simulink model "Impl_None"  (R2026b)
settings: Solver=VariableStepAuto
undefined symbols (not defined in the file or in its folder): P, Ts
libraries: fl_lib x7, simulink x1, ee_lib x1
settings Model: Creator=aomar  LastModifiedBy=aomar

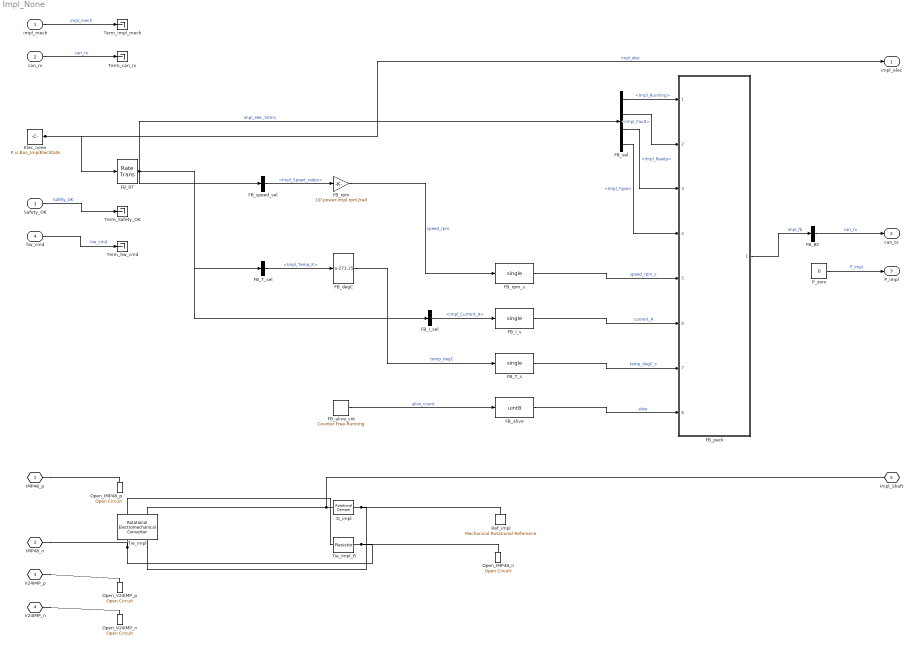
== system Impl_None ==
  impl_mech : Inport  OutDataTypeStr=Bus: Bus_ImplMechState  SampleTime=Ts.ctrl
  can_rx : Inport  Port=2  OutDataTypeStr=Bus: Bus_Can1_McuSlow  SampleTime=Ts.can_slow
  Safety_OK : Inport  Port=3  OutDataTypeStr=boolean  SampleTime=Ts.safety
  hw_cmd : Inport  Port=4  OutDataTypeStr=Bus: Bus_PowerHwCmd  SampleTime=Ts.base
  D_impl : fl_lib/Mechanical/Rotational Elements/Rotational Damper  D=P.power.impl.D_none N*m*s/rad  w_specify=off  w_priority=None  w=0 rad/s  w_nominal_specify=off  w_nominal_value=1  w_nominal_unit=rad/s  t_specify=off  t_priority=None  t=0 N*m  t_nominal_specify=off  t_nominal_value=1  t_nominal_unit=N*m
  Elec_none : Constant  Value=P.ic.Bus_ImplElecState  OutDataTypeStr=Bus: Bus_ImplElecState  SampleTime=Ts.impl_ctrl
  FB_BC : BusCreator  Inputs=1  OutDataTypeStr=Bus: Bus_Can1_Impl  NonVirtualBus=on
      settings: InheritFromInputs=off
  FB_I_s : DataTypeConversion  OutDataTypeStr=single  SaturateOnIntegerOverflow=off  RndMeth=Floor
  FB_I_sel : BusSelector  OutputSignals=Impl_Current_A
  FB_RT : RateTransition  OutPortSampleTime=Ts.can_slow
  FB_T_s : DataTypeConversion  OutDataTypeStr=single  SaturateOnIntegerOverflow=off  RndMeth=Floor
  FB_T_sel : BusSelector  OutputSignals=Impl_Temp_K
  FB_alive : DataTypeConversion  OutDataTypeStr=uint8  SaturateOnIntegerOverflow=off  RndMeth=Floor
  FB_alive_cnt : simulink/Sources/Counter Free-Running  NumBits=8  tsamp=Ts.can_slow
  FB_degC : Bias  Bias=-273.15  SaturateOnIntegerOverflow=off
  FB_pack : Subsystem  ReferencedSubsystem=implfb_can_pack
  FB_rpm : Gain  Gain=1/P.power.impl.rpm2rad
  FB_rpm_s : DataTypeConversion  OutDataTypeStr=single  SaturateOnIntegerOverflow=off  RndMeth=Floor
  FB_sel : BusSelector  OutputSignals=Impl_Running,Impl_Fault,Impl_Ready,Impl_Type
  FB_speed_sel : BusSelector  OutputSignals=Impl_Speed_radps
  Open_IMP48_n : fl_lib/Electrical/Electrical Elements/Open Circuit  v_specify=off  v_priority=None  v=0 V  v_nominal_specify=off  v_nominal_value=1  v_nominal_unit=V
      settings: LibrarySourceBlock=|
      | ee_lib/Connectors &
      | References/Open Circuit
  Open_IMP48_p : fl_lib/Electrical/Electrical Elements/Open Circuit  v_specify=off  v_priority=None  v=0 V  v_nominal_specify=off  v_nominal_value=1  v_nominal_unit=V
      settings: LibrarySourceBlock=|
      | ee_lib/Connectors &
      | References/Open Circuit
  Open_V24IMP_n : fl_lib/Electrical/Electrical Elements/Open Circuit  v_specify=off  v_priority=None  v=0 V  v_nominal_specify=off  v_nominal_value=1  v_nominal_unit=V
      settings: LibrarySourceBlock=|
      | ee_lib/Connectors &
      | References/Open Circuit
  Open_V24IMP_p : fl_lib/Electrical/Electrical Elements/Open Circuit  v_specify=off  v_priority=None  v=0 V  v_nominal_specify=off  v_nominal_value=1  v_nominal_unit=V
      settings: LibrarySourceBlock=|
      | ee_lib/Connectors &
      | References/Open Circuit
  P_zero : Constant  Value=0  OutDataTypeStr=double  SampleTime=Ts.base
  Ref_impl : fl_lib/Mechanical/Rotational Elements/Mechanical Rotational Reference
  Term_Safety_OK : Terminator
  Term_can_rx : Terminator
  Term_hw_cmd : Terminator
  Term_impl_mech : Terminator
  Tie_impl : fl_lib/Electrical/Electrical Elements/Rotational Electromechanical Converter  K=P.drive.tie.K V*s/rad  i_specify=off  i_priority=None  i=0 A  i_nominal_specify=off  i_nominal_value=1  i_nominal_unit=A  v_specify=off  v_priority=None  v=0 V  v_nominal_specify=off  v_nominal_value=1  v_nominal_unit=V  t_specify=off  t_priority=None  t=0 N*m  t_nominal_specify=off  t_nominal_value=1  t_nominal_unit=N*m  w_specify=off  w_priority=None  w=0 rad/s  w_nominal_specify=off  w_nominal_value=1  w_nominal_unit=rad/s
  Tie_impl_R : ee_lib/Passive/Resistor  R=P.drive.tie.R Ohm  enable_R_tol=ee.enum.toleranceApplication.none  R_tol=5  tol_distribution=ee.enum.toleranceDistribution.uniform  nSigma=4  enable_operating_limits=ee.enum.enable.no  operating_limit_action=ee.enum.passive.reportOpLim.warn  power_rating=1 W  max_working_voltage=100 V  noise_mode=ee.enum.sources.noise.Disabled  Tdevice=25 degC  sample_time=1e-3 s  repeatability=ee.enum.ic.repeatability.notRepeatable  user_seed=0  auto_seed=3191729647  power_derating_T1=70 degC  power_derating_T2=155 degC  operating_temperature_range_vec=[-50, 150] degC  alpha=3.93e-3 1/K  Tmeas=25 degC  thermal_mass=100 J/K  temperature_specify=off  temperature_priority=High  temperature=298.15 K  temperature_nominal_specify=off  temperature_nominal_value=1  temperature_nominal_unit=K
  IMP48_p : PMIOPort  Side=Left  ConnectionType=Connection: foundation.electrical.electrical
  IMP48_n : PMIOPort  Port=2  Side=Left  ConnectionType=Connection: foundation.electrical.electrical
  V24IMP_p : PMIOPort  Port=3  Side=Left  ConnectionType=Connection: foundation.electrical.electrical
  V24IMP_n : PMIOPort  Port=4  Side=Left  ConnectionType=Connection: foundation.electrical.electrical
  Impl_Shaft : PMIOPort  Port=5  Side=Right  ConnectionType=Connection: foundation.mechanical.rotational.rotational
  impl_elec : Outport  OutDataTypeStr=Bus: Bus_ImplElecState
  can_tx : Outport  Port=2  OutDataTypeStr=Bus: Bus_Can1_Impl
  P_impl : Outport  Port=3  OutDataTypeStr=double
  wires:
  impl_mech/1 -> Term_impl_mech/1  "impl_mech"
  can_rx/1 -> Term_can_rx/1  "can_rx"
  Elec_none/1 -> impl_elec/1, FB_RT/1  "impl_elec"
  Safety_OK/1 -> Term_Safety_OK/1  "Safety_OK"
  hw_cmd/1 -> Term_hw_cmd/1  "hw_cmd"
  FB_RT/1 -> FB_I_sel/1, FB_T_sel/1, FB_sel/1, FB_speed_sel/1  "impl_elec_50ms"
  FB_speed_sel/1 -> FB_rpm/1  "<Impl_Speed_radps>"
  FB_T_sel/1 -> FB_degC/1  "<Impl_Temp_K>"
  FB_rpm/1 -> FB_rpm_s/1  "speed_rpm"
  FB_alive_cnt/1 -> FB_alive/1  "alive_count"
  FB_degC/1 -> FB_T_s/1  "temp_degC"
  FB_I_sel/1 -> FB_I_s/1  "<Impl_Current_A>"
  FB_rpm_s/1 -> FB_pack/5  "speed_rpm_s"
  FB_I_s/1 -> FB_pack/6  "current_A"
  FB_T_s/1 -> FB_pack/7  "temp_degC_s"
  FB_alive/1 -> FB_pack/8  "alive"
  FB_sel/1 -> FB_pack/1  "<Impl_Running>"
  FB_sel/2 -> FB_pack/2  "<Impl_Fault>"
  FB_sel/3 -> FB_pack/3  "<Impl_Ready>"
  FB_sel/4 -> FB_pack/4  "<Impl_Type>"
  FB_pack/1 -> FB_BC/1  "impl_fb"
  FB_BC/1 -> can_tx/1  "can_tx"
  P_zero/1 -> P_impl/1  "P_impl"
  connections:
  D_impl/LConn1 -- Tie_impl/LConn2 -- Impl_Shaft/RConn1
  D_impl/RConn1 -- Tie_impl/RConn2 -- Ref_impl/LConn1
  Tie_impl/RConn1 -- IMP48_n/RConn1 -- Tie_impl_R/RConn1 -- Open_IMP48_n/LConn1
  IMP48_p/RConn1 -- Open_IMP48_p/LConn1
  V24IMP_n/RConn1 -- Open_V24IMP_n/LConn1
  V24IMP_p/RConn1 -- Open_V24IMP_p/LConn1
  Tie_impl/LConn1 -- Tie_impl_R/LConn1
